simulink model "Bidirectional_Half_Bridge_DCDC"  (R2021a)
settings: Solver=VariableStepAuto  StartTime=0.0  StopTime=10.0  RelTol=1e-3
libraries: spsSeriesRLCBranchLib x3, spsCurrentMeasurementLib x2, spsDCVoltageSourceLib x2, spsMosfetLib x2, spsVoltageMeasurementLib x2, pid_lib x1, spsPWMGenerator2LevelLib x1, simulink x1, spspowerguiLib x1
settings Model: Creator=45276  LastModifiedBy=45276

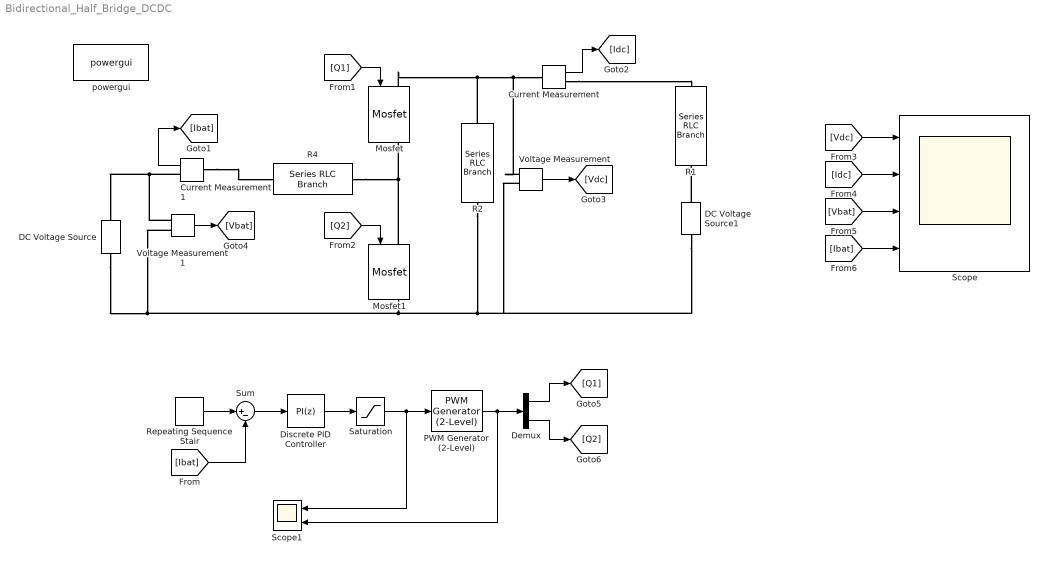
== system Bidirectional_Half_Bridge_DCDC ==
  Current Measurement : spsCurrentMeasurementLib/Current Measurement  PhasorSimulation=off  OutputType=Complex  PSBequivalent=0
  Current Measurement1 : spsCurrentMeasurementLib/Current Measurement  PhasorSimulation=off  OutputType=Complex  PSBequivalent=0
  DC Voltage Source : spsDCVoltageSourceLib/DC Voltage Source  Amplitude=18  Measurements=None
  DC Voltage Source1 : spsDCVoltageSourceLib/DC Voltage Source  Amplitude=30  Measurements=None
  Demux : Demux  Outputs=2
  Discrete PID Controller : pid_lib/PID Controller  Controller=PI  Form=Parallel  TimeDomain=Discrete-time  UseExternalTs=off  SampleTime=1/20e3  IntegratorMethod=Forward Euler  FilterMethod=Forward Euler  ControllerParametersSource=internal  P=5  I=100  D=0  UseFilter=on  N=100  TunerSelectOption=Transfer Function Based (PID Tuner App)  InitialConditionSource=internal  InitialConditionForIntegrator=0  InitialConditionForFilter=0  DifferentiatorICPrevScaledInput=0  ExternalReset=none  TrackingMode=off  Kt=1  LimitOutput=off  SatLimitsSource=internal  UpperSaturationLimit=inf  LowerSaturationLimit=-inf  LinearizeAsGain=off  AntiWindupMode=none  Kb=1  POutMin=[]  POutMax=[]  IOutMin=[]  IOutMax=[]  DOutMin=[]  DOutMax=[]  NOutMin=[]  NOutMax=[]  SumOutMin=[]  SumOutMax=[]  SaturationOutMin=[]  SaturationOutMax=[]  PParamMin=[]  PParamMax=[]  IParamMin=[]  IParamMax=[]  DParamMin=[]  DParamMax=[]  NParamMin=[]  NParamMax=[]  KbParamMin=[]  KbParamMax=[]  KtParamMin=[]  KtParamMax=[]  KbOutMin=[]  KbOutMax=[]  KtOutMin=[]  KtOutMax=[]  IntegratorOutMin=[]  IntegratorOutMax=[]  FilterOutMin=[]  FilterOutMax=[]  SumI1OutMin=[]  SumI1OutMax=[]  SumI2OutMin=[]  SumI2OutMax=[]  SumI3OutMin=[]  SumI3OutMax=[]  SumI4OutMin=[]  SumI4OutMax=[]  SumDOutMin=[]  SumDOutMax=[]  DifferentiatorOutMin=[]  DifferentiatorOutMax=[]  FilterDiffOutCoefMin=[]  FilterDiffOutCoefMax=[]  ReciprocalOutMin=[]  ReciprocalOutMax=[]  SumDenOutMin=[]  SumDenOutMax=[]  SumNumOutMin=[]  SumNumOutMax=[]  DivideOutMin=[]  DivideOutMax=[]  UdiffTsProdOutMin=[]  UdiffTsProdOutMax=[]  NTsProdOutMin=[]  NTsProdOutMax=[]  UintegralTsProdOutMin=[]  UintegralTsProdOutMax=[]  UngainTsProdOutMin=[]  UngainTsProdOutMax=[]  IntegratorContinuousStateAttributes=''  IntegratorStateMustResolveToSignalObject=off  IntegratorRTWStateStorageClass=Auto  FilterContinuousStateAttributes=''  FilterStateMustResolveToSignalObject=off  FilterRTWStateStorageClass=Auto  ParallelPVariant=InternalParameters  IdealPVariant=Disabled  IVariant=InternalParameters  DVariant=Disabled  IntegratorVariant=Discrete  SatVariant=Disabled  AWVariant=Passthrough  PCopyVariant=Disabled  TRVariant=Disabled  FdbkBlocksVariant=Forward  IdealPFdbkVariant=Disabled  SatFdbkVariant=Disabled  DerivativeFilterVariant=Disabled  NVariant=Disabled  NCopyVariant=Disabled_SignalSpec  FilterICVariant=Disabled  IntegratorICVariant=InternalICs  ExternalResetVariant=Disabled  TRSumVariant=Passthrough  SumFdbkVariant=Disabled  SumVariant=Sum_PI  TsampFilterVariant=InternalTs  TsampNgainVariant=Passthrough  TsampIntegralVariant=Passthrough  ExternalSaturationOutDataTypeStr=Inherit: Same as second input
  Mosfet : spsMosfetLib/Mosfet  Ron=0.1  Lon=0  Rd=0.01  Vfd=0  IC=0  Rs=1e5  Cs=inf  Measurements=on
  Mosfet1 : spsMosfetLib/Mosfet  Ron=0.1  Lon=0  Rd=0.01  Vfd=0  IC=0  Rs=1e5  Cs=inf  Measurements=on
  PWM Generator (2-Level) : spsPWMGenerator2LevelLib/PWM Generator (2-Level)  ModulatorType=Single-phase half-bridge (2 pulses)  ModulatorMode=Unsynchronized  Fc=20000  Pc=90  nF=27  MinMax="[ -1  1 ]"  SamplingTechnique=Natural  ModulatingSignals=off  m=0.8  Freq=60  Phase=0  Ts=0  ShowCarrierOutport=off
  R1 : spsSeriesRLCBranchLib/Series RLC Branch  LConnTagsString=__new0  RConnTagsString=__new0  BranchType=R  Resistance=0.1  Inductance=1e-3  SetiL0=off  InitialCurrent=0  Capacitance=1e-6  Setx0=off  InitialVoltage=0  Measurements=None
  R2 : spsSeriesRLCBranchLib/Series RLC Branch  LConnTagsString=__new0  RConnTagsString=__new0  BranchType=RC  Resistance=1e-3  Inductance=1e-3  SetiL0=off  InitialCurrent=0  Capacitance=4.7e-6  Setx0=off  InitialVoltage=0  Measurements=None
  R4 : spsSeriesRLCBranchLib/Series RLC Branch  LConnTagsString=__new0  RConnTagsString=__new0  BranchType=RL  Resistance=1e-3  Inductance=1e-3  SetiL0=off  InitialCurrent=0  Capacitance=1e-6  Setx0=off  InitialVoltage=0  Measurements=None
  Repeating Sequence Stair : simulink/Sources/Repeating Sequence Stair  OutValues=[3 0.5 4 2 1].'  tsamp=0.2  OutMin=[]  OutMax=[]  OutDataTypeStr=double  OutputDataTypeScalingMode=double  OutDataType=fixdt(0,8)  ConRadixGroup=Best Precision: Vector-wise  OutScaling=2^-12
  Saturation : Saturate  UpperLimit=0.9  LowerLimit=0
  Scope : Scope  NumInputPorts=4
  Scope1 : Scope  NumInputPorts=2
  Sum : Sum  Inputs=|+-
  Voltage Measurement : spsVoltageMeasurementLib/Voltage Measurement  PhasorSimulation=off  OutputType=Complex  PSBequivalent=0
  Voltage Measurement1 : spsVoltageMeasurementLib/Voltage Measurement  PhasorSimulation=off  OutputType=Complex  PSBequivalent=0
  powergui : spspowerguiLib/powergui  Priority=1  SimulationMode=Discrete  SampleTime=1e-06  frequency=60  Iterations=50  frequencyindice=0  Pbase=100e6  ErrMax=1e-4  UnitsV=kV  UnitsW=MW  buscounter=0  FunctionMessages=off  echomessages=off  EnableUseOfTLC=off  CurrentSourceSwitches=off  DisableSnubberDevices=off  DisableRonSwitches=off  DisableVfSwitches=off  DisplayEquations=off  AutomaticDiscreteSolvers=off  SolverType=Tustin/Backward Euler (TBE)  Interpol=off  ExternalGateDelay=off  methode=off  Ts=100  x0status=blocks  SPID=on  SwTol=0  HookPort=off  NonlinearTolerance=1e-4  nMaxIteration=100  ContinueOnMaxIteration=off  RestoreLinks=warning  ResistiveCurrentMeasurement=off  Frange=[0:2:500]  Ylog=off  Xlog=on  ShowGrid=off  save=off  variable=ZData  structure=0  ZoomFFT=off  StartTime=0.0  cycles=1  DisplayStyle=1  fundamental=60  FreqAxis=off  MaxFrequency=1000  frequencyindicesteady=1  RmsSteady=1  display=off
  wires:
  Discrete PID Controller/1 -> Saturation/1
  Saturation/1 -> Scope1/1, PWM Generator (2-Level)/1
  Sum/1 -> Discrete PID Controller/1
  Repeating Sequence Stair/1 -> Sum/1
  [Ibat] -> Sum/2
  PWM Generator (2-Level)/1 -> Scope1/2, Demux/1
  Current Measurement1/1 -> [Ibat]
  Current Measurement/1 -> [Idc]
  Voltage Measurement/1 -> [Vdc]
  Voltage Measurement1/1 -> [Vbat]
  [Q1] -> Mosfet/1
  [Q2] -> Mosfet1/1
  Demux/1 -> [Q1]
  Demux/2 -> [Q2]
  [Vdc] -> Scope/1
  [Idc] -> Scope/2
  [Vbat] -> Scope/3
  [Ibat] -> Scope/4
  connections:
  DC Voltage Source1/RConn1 -- R1/LConn1
  R2/RConn1 -- Voltage Measurement/LConn1 -- Current Measurement/LConn1 -- Mosfet/LConn1
  Current Measurement/RConn1 -- R1/RConn1
  R2/LConn1 -- DC Voltage Source1/LConn1 -- Voltage Measurement/LConn2 -- Mosfet1/RConn1 -- Voltage Measurement1/LConn2 -- DC Voltage Source/LConn1
  Voltage Measurement1/LConn1 -- Current Measurement1/RConn1 -- DC Voltage Source/RConn1
  Mosfet1/LConn1 -- R4/LConn1 -- Mosfet/RConn1
  Current Measurement1/LConn1 -- R4/RConn1
